simulink model "AFC2_F_trainscg_15_15_15_15_controller_ep_500_Nor_20250717"  (R2021a)
settings: Solver=VariableStepAuto  StartTime=0.0  StopTime=10.0  RelTol=1e-3
libraries: neural x66
(part 3 of 3)

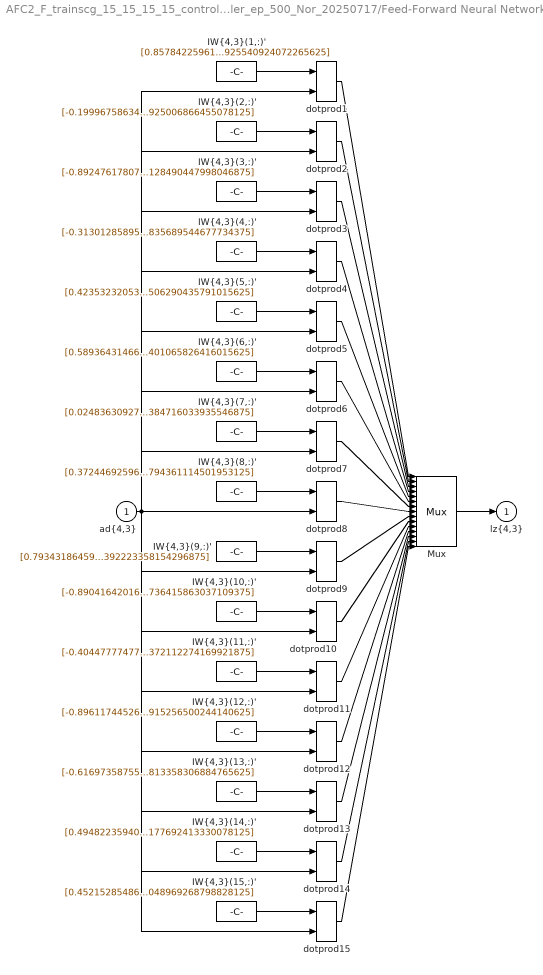
== system AFC2_F_trainscg_15_15_15_15_controller_ep_500_Nor_20250717/Feed-Forward Neural Network/Layer 4/LW{4,3} ==
  "ad{4,3}" : Inport  PortDimensions=15
      mask Display: e = 0.06;c1 = [120 230 180]/255;c2 = ([120 230 180]+0)/(256+128);c3 = ([120 230 180]+128)/(256+128);patch([0 1 1 0],[0 0 1 1],c1);patch([0 1 1 1-e 1-e 0+e],[0 0 1 1-e 0+e 0+e],c2);patch([0 0 1 1-e 0+e 0+e],[0 1 1 1-e 1-e 0+e],c3);plot([0 1 1 0 0],[0 0 1 1 0]);
  "IW{4,3}(1,:)'" : Constant  Value=[0.85784225961529048110065787113853730261325836181640625;0.755479109208128551955496732261963188648223876953125;0.050445139131901829687709692962016561068594455718994140625;-0.426758953537573315628605996607802808284759521484375;0.68113585156923750485447044411557726562023162841796875;0.548222043336579201167069186340086162090301513671875;-0.09920996923674353651367852080511511303484439849853515625;-0.210186876811422396205131235547014512121677398681640625;-0.7277467957558354516578447146457619965076446533203125;0.654091436703768014382376350113190710544586181640625;0.9937004291498972019525126597727648913860321044921875;0.862223254974441299935961069422774016857147216796875;0.4407088843135629208092041153577156364917755126953125;-0.1026007594675311385135074715435621328651905059814453125;0.33596462844713192996692896485910750925540924072265625]
      mask Display: e = 0.06;c1 = [120 150 230]/255;c2 = ([120 150 230]+0)/383;c3 = ([120 150 230]+128)/383;patch([0 1 1 0],[0 0 1 1],c1);patch([0 1 1 1-e 1-e 0+e],[0 0 1 1-e 0+e 0+e],c2);patch([0 0 1 1-e 0+e 0+e],[0 1 1 1-e 1-e 0+e],c3);plot([0 1 1 0 0],[0 0 1 1 0]);disp('weights');
  "IW{4,3}(10,:)'" : Constant  Value=[-0.8904164201605351269819266235572285950183868408203125;0.67793926298775630812087911181151866912841796875;-0.732992210954486633767146486206911504268646240234375;-0.948285057833720745890104808495379984378814697265625;-0.85589678168697302940159943318576551973819732666015625;0.76567535318746748895790688038687221705913543701171875;-0.1853631538863742544975821147090755403041839599609375;0.768810196191384687125491836923174560070037841796875;-0.20373816257141508234695947976433672010898590087890625;-0.80925461474435689268602800439111888408660888671875;-0.127630088537103336676636899937875568866729736328125;-0.5958498069031368249426350303110666573047637939453125;0.46277413232386610530966208898462355136871337890625;-0.89931988538168672331352127002901397645473480224609375;-0.6949987259950594076229890561080537736415863037109375]
      mask Display: e = 0.06;c1 = [120 150 230]/255;c2 = ([120 150 230]+0)/383;c3 = ([120 150 230]+128)/383;patch([0 1 1 0],[0 0 1 1],c1);patch([0 1 1 1-e 1-e 0+e],[0 0 1 1-e 0+e 0+e],c2);patch([0 0 1 1-e 0+e 0+e],[0 1 1 1-e 1-e 0+e],c3);plot([0 1 1 0 0],[0 0 1 1 0]);disp('weights');
  "IW{4,3}(11,:)'" : Constant  Value=[-0.404477774774269993596220729159540496766567230224609375;-0.1346711516861960056257174755955929867923259735107421875;-1.0044851640110368240499383318820036947727203369140625;-0.10694362204521722092831481631947099231183528900146484375;-0.219228550864126792152575262662139721214771270751953125;0.784925570810754980044521289528347551822662353515625;-0.4494260973686199367449489727732725441455841064453125;0.408791248658470995902547429068363271653652191162109375;-0.0217524709232971014127855369224562309682369232177734375;-0.70697111014115987526196249746135435998439788818359375;0.65325901323778357010496620205231010913848876953125;-0.0922130686389561748939058816176839172840118408203125;-0.2799379158284567292724887010990642011165618896484375;-0.56685462762244764878261094054323621094226837158203125;-0.96075786646883187813728000037372112274169921875]
      mask Display: e = 0.06;c1 = [120 150 230]/255;c2 = ([120 150 230]+0)/383;c3 = ([120 150 230]+128)/383;patch([0 1 1 0],[0 0 1 1],c1);patch([0 1 1 1-e 1-e 0+e],[0 0 1 1-e 0+e 0+e],c2);patch([0 0 1 1-e 0+e 0+e],[0 1 1 1-e 1-e 0+e],c3);plot([0 1 1 0 0],[0 0 1 1 0]);disp('weights');
  "IW{4,3}(12,:)'" : Constant  Value=[-0.89611744526934866694745096538099460303783416748046875;-0.05990124759827260281230820737619069404900074005126953125;0.11155310785038198562180156159229227341711521148681640625;0.292599689876200608207312825470580719411373138427734375;0.301985443034309575249807267027790658175945281982421875;0.0822405223753759628824155925030936487019062042236328125;0.433314698716638968534198284032754600048065185546875;-0.9856862277475759714917558085289783775806427001953125;0.30650451235397735416654541040770709514617919921875;0.27569206039626925619501207620487548410892486572265625;-0.21093063153393298847504411241970956325531005859375;-0.1441781603596583583026813357719220221042633056640625;-0.09332817707907252458010560758339124731719493865966796875;0.60984306977241542480072666876367293298244476318359375;-0.133728085119795780943974250476458109915256500244140625]
      mask Display: e = 0.06;c1 = [120 150 230]/255;c2 = ([120 150 230]+0)/383;c3 = ([120 150 230]+128)/383;patch([0 1 1 0],[0 0 1 1],c1);patch([0 1 1 1-e 1-e 0+e],[0 0 1 1-e 0+e 0+e],c2);patch([0 0 1 1-e 0+e 0+e],[0 1 1 1-e 1-e 0+e],c3);plot([0 1 1 0 0],[0 0 1 1 0]);disp('weights');
  "IW{4,3}(13,:)'" : Constant  Value=[-0.6169735875510138356503375689499080181121826171875;0.12196946325811171274455801949443412013351917266845703125;-0.394484793782070075618406690409756265580654144287109375;0.042406510402860718433881714872768498025834560394287109375;0.88124737799676766680789796737371943891048431396484375;0.21174326427215739432341479187016375362873077392578125;-0.433210125755401354030738048095372505486011505126953125;0.36155480448124122094810672933817841112613677978515625;0.8992327827721648958458899869583547115325927734375;0.71234708636273236237457240349613130092620849609375;0.226949763410523974727084350888617336750030517578125;0.93210549922399810185424939845688641071319580078125;-0.2258655976427387523930434554131352342665195465087890625;-0.93860108197167602117616524992627091705799102783203125;0.66555016185605231360256084371940232813358306884765625]
      mask Display: e = 0.06;c1 = [120 150 230]/255;c2 = ([120 150 230]+0)/383;c3 = ([120 150 230]+128)/383;patch([0 1 1 0],[0 0 1 1],c1);patch([0 1 1 1-e 1-e 0+e],[0 0 1 1-e 0+e 0+e],c2);patch([0 0 1 1-e 0+e 0+e],[0 1 1 1-e 1-e 0+e],c3);plot([0 1 1 0 0],[0 0 1 1 0]);disp('weights');
  "IW{4,3}(14,:)'" : Constant  Value=[0.49482235940801666540522774084820412099361419677734375;-0.4633443699893644573961637433967553079128265380859375;0.8250812426062681392835429505794309079647064208984375;-0.25538462229765335198550246786908246576786041259765625;0.471927834000104462486291367895319126546382904052734375;-0.90296620984852771218953648713068105280399322509765625;0.79233153905017028595381134437047876417636871337890625;-0.2246600162756056950907890268354094587266445159912109375;0.450286481803449323280119642731733620166778564453125;1.065736521854187213165232606115750968456268310546875;0.63728147016441827332755565294064581394195556640625;0.240110108266947452904105375637300312519073486328125;0.54537100983026076672643966958275996148586273193359375;0.49952096707471638215025677709490992128849029541015625;0.2023225447090571116337542889596079476177692413330078125]
      mask Display: e = 0.06;c1 = [120 150 230]/255;c2 = ([120 150 230]+0)/383;c3 = ([120 150 230]+128)/383;patch([0 1 1 0],[0 0 1 1],c1);patch([0 1 1 1-e 1-e 0+e],[0 0 1 1-e 0+e 0+e],c2);patch([0 0 1 1-e 0+e 0+e],[0 1 1 1-e 1-e 0+e],c3);plot([0 1 1 0 0],[0 0 1 1 0]);disp('weights');
  "IW{4,3}(15,:)'" : Constant  Value=[0.4521528548690147975008812863961793482303619384765625;0.498047205681803717425282229669392108917236328125;0.9807228794230840041024066522368229925632476806640625;0.87426933268312456704052237910218536853790283203125;-0.034445771129767828455658928987759281881153583526611328125;0.7903040721398146839504761373973451554775238037109375;0.653157784627120374665310009731911122798919677734375;-0.133542756460722056299772475540521554648876190185546875;-0.15248315354482377959044470117078162729740142822265625;0.1597864707538303452594163900357671082019805908203125;0.7724700781252129555554120088345371186733245849609375;0.3907799038360071364195391652174293994903564453125;0.4685422113718786807368132940609939396381378173828125;-0.84392316757664620485712703157332725822925567626953125;0.040266212651737638694715570863991160877048969268798828125]
      mask Display: e = 0.06;c1 = [120 150 230]/255;c2 = ([120 150 230]+0)/383;c3 = ([120 150 230]+128)/383;patch([0 1 1 0],[0 0 1 1],c1);patch([0 1 1 1-e 1-e 0+e],[0 0 1 1-e 0+e 0+e],c2);patch([0 0 1 1-e 0+e 0+e],[0 1 1 1-e 1-e 0+e],c3);plot([0 1 1 0 0],[0 0 1 1 0]);disp('weights');
  "IW{4,3}(2,:)'" : Constant  Value=[-0.1999675863494781713480819007600075565278530120849609375;0.164304483540531898189129833554034121334552764892578125;0.294920972712406748161839686872554011642932891845703125;0.60163861334048807094632138614542782306671142578125;0.689838390875554097192434710450470447540283203125;-0.1725769714967674561822974510505446232855319976806640625;-0.588657896836348282221251793089322745800018310546875;-0.01143321893140521704201884034546310431323945522308349609375;0.62470927507009055279496578805265016853809356689453125;-0.731227381749264271348920374293811619281768798828125;0.1070831469910651367882792328600771725177764892578125;-0.61843070398175559176934257266111671924591064453125;-0.30635878824157902755587201681919395923614501953125;0.371878731756418778875428188257501460611820220947265625;-0.00077214337368226274201099545990700789843685925006866455078125]
      mask Display: e = 0.06;c1 = [120 150 230]/255;c2 = ([120 150 230]+0)/383;c3 = ([120 150 230]+128)/383;patch([0 1 1 0],[0 0 1 1],c1);patch([0 1 1 1-e 1-e 0+e],[0 0 1 1-e 0+e 0+e],c2);patch([0 0 1 1-e 0+e 0+e],[0 1 1 1-e 1-e 0+e],c3);plot([0 1 1 0 0],[0 0 1 1 0]);disp('weights');
  "IW{4,3}(3,:)'" : Constant  Value=[-0.89247617807962276170741233727312646806240081787109375;-0.86100607739435730536570190452039241790771484375;-0.419841694707571988498528980926494114100933074951171875;0.79221535087837258171106213922030292451381683349609375;-0.2607743664207731182358429578016512095928192138671875;0.941656695538196419903442802024073898792266845703125;0.7993019809456687330140312042203731834888458251953125;0.369587645665073905032471657250425778329372406005859375;-0.395000547100446908199700146724353544414043426513671875;-0.88802182418189712365119703463278710842132568359375;0.030916909680651638581139195594005286693572998046875;-0.482835497162455329345220889081247150897979736328125;0.03380749306426929223778898858654429204761981964111328125;0.84153428281462883120411788695491850376129150390625;-0.5796887383710351837606822300585918128490447998046875]
      mask Display: e = 0.06;c1 = [120 150 230]/255;c2 = ([120 150 230]+0)/383;c3 = ([120 150 230]+128)/383;patch([0 1 1 0],[0 0 1 1],c1);patch([0 1 1 1-e 1-e 0+e],[0 0 1 1-e 0+e 0+e],c2);patch([0 0 1 1-e 0+e 0+e],[0 1 1 1-e 1-e 0+e],c3);plot([0 1 1 0 0],[0 0 1 1 0]);disp('weights');
  "IW{4,3}(4,:)'" : Constant  Value=[-0.31301285895226749200759286395623348653316497802734375;0.85004642369605420970657405632664449512958526611328125;-0.6971020802553307138538229992263950407505035400390625;0.1950664900871264817450168038703850470483303070068359375;0.2070968237721194371570021530715166591107845306396484375;1.0010743549489260484364194780937395989894866943359375;0.5251710787464538565672000913764350116252899169921875;0.68577610833234003973046810642699711024761199951171875;-0.48133678245497069081437757631647400557994842529296875;-0.8315058953706808697603491964400745928287506103515625;-0.3386358680194658798967566326609812676906585693359375;0.7957313696805983216364666077424772083759307861328125;0.1133892640242037952447162751923315227031707763671875;0.59421402291022207275972277784603647887706756591796875;0.1432314508081782289394823237671516835689544677734375]
      mask Display: e = 0.06;c1 = [120 150 230]/255;c2 = ([120 150 230]+0)/383;c3 = ([120 150 230]+128)/383;patch([0 1 1 0],[0 0 1 1],c1);patch([0 1 1 1-e 1-e 0+e],[0 0 1 1-e 0+e 0+e],c2);patch([0 0 1 1-e 0+e 0+e],[0 1 1 1-e 1-e 0+e],c3);plot([0 1 1 0 0],[0 0 1 1 0]);disp('weights');
  "IW{4,3}(5,:)'" : Constant  Value=[0.423532320530276729098062560296966694295406341552734375;0.5994190748139638369451631660922430455684661865234375;-0.149139137079837669208615125171490944921970367431640625;0.76802951129515850681173105840571224689483642578125;0.6884912802328846392896366523928008973598480224609375;0.66321777623028455028730832054861821234226226806640625;0.764972614800595973605368271819315850734710693359375;0.17128163825504449935266393367783166468143463134765625;-0.450420586012070078840707765266415663063526153564453125;-0.6912346804131728195130790481925942003726959228515625;-0.139996403213207276650109633919782936573028564453125;0.1867237207722178826685421881848014891147613525390625;-0.687009561771910970406906926655210554599761962890625;0.391552682266078144746046518775983713567256927490234375;-0.75476930316581614111015596790821291506290435791015625]
      mask Display: e = 0.06;c1 = [120 150 230]/255;c2 = ([120 150 230]+0)/383;c3 = ([120 150 230]+128)/383;patch([0 1 1 0],[0 0 1 1],c1);patch([0 1 1 1-e 1-e 0+e],[0 0 1 1-e 0+e 0+e],c2);patch([0 0 1 1-e 0+e 0+e],[0 1 1 1-e 1-e 0+e],c3);plot([0 1 1 0 0],[0 0 1 1 0]);disp('weights');
  "IW{4,3}(6,:)'" : Constant  Value=[0.589364314667610411646592183387838304042816162109375;-0.4281062871592735685766228925785981118679046630859375;-0.2750814383625079795336887400480918586254119873046875;0.88746308239158278041713856509886682033538818359375;0.86700321701421056985736868227832019329071044921875;-0.2222324481751429825493460157304070889949798583984375;-0.4300995639503575329598561438615433871746063232421875;0.1494743217128160495121846906840801239013671875;-0.24861571998082343526448312331922352313995361328125;-0.351560159411901995696325684548355638980865478515625;-0.0163874927925105051684795398614369332790374755859375;0.0076801636936958406209896565997041761875152587890625;0.1241120911235495949398455195478163659572601318359375;-0.781331520951308533540213829837739467620849609375;0.342332465977305933080288014025427401065826416015625]
      mask Display: e = 0.06;c1 = [120 150 230]/255;c2 = ([120 150 230]+0)/383;c3 = ([120 150 230]+128)/383;patch([0 1 1 0],[0 0 1 1],c1);patch([0 1 1 1-e 1-e 0+e],[0 0 1 1-e 0+e 0+e],c2);patch([0 0 1 1-e 0+e 0+e],[0 1 1 1-e 1-e 0+e],c3);plot([0 1 1 0 0],[0 0 1 1 0]);disp('weights');
  "IW{4,3}(7,:)'" : Constant  Value=[0.0248363092718685181392590521909369272179901599884033203125;0.0887981324634880830881655811026575975120067596435546875;0.63494523170573557990792323835194110870361328125;0.09832708137094652023346696978478576056659221649169921875;0.4971322170728871281397687198477797210216522216796875;0.1245748260428689857537420948574435897171497344970703125;0.34652832367269181812474698745063506066799163818359375;-0.236815899621558079157779275192297063767910003662109375;0.078844710400133022343283073496422730386257171630859375;-0.52511982239588295140464424548554234206676483154296875;-0.8579258321740945714140025302185676991939544677734375;0.225619177671118276151673853746615350246429443359375;0.39622423096519876484222777435206808149814605712890625;0.0293784494319486687297082738723474903963506221771240234375;0.2333234784644419856913799549147370271384716033935546875]
      mask Display: e = 0.06;c1 = [120 150 230]/255;c2 = ([120 150 230]+0)/383;c3 = ([120 150 230]+128)/383;patch([0 1 1 0],[0 0 1 1],c1);patch([0 1 1 1-e 1-e 0+e],[0 0 1 1-e 0+e 0+e],c2);patch([0 0 1 1-e 0+e 0+e],[0 1 1 1-e 1-e 0+e],c3);plot([0 1 1 0 0],[0 0 1 1 0]);disp('weights');
  "IW{4,3}(8,:)'" : Constant  Value=[0.37244692596808182116774332826025784015655517578125;0.9695524739412195724952425734954886138439178466796875;0.5605916416882192887527480706921778619289398193359375;0.4567736491887133265521470093517564237117767333984375;-0.58644708412978996392439512419514358043670654296875;-0.5066256047238415494149421647307462990283966064453125;0.32855980883610147458284700405783951282501220703125;-0.087150798296506071238809454371221363544464111328125;0.1238403085319534913111283458420075476169586181640625;-0.9766380177393207961955567952827550470829010009765625;0.7754784310654321277667122558341361582279205322265625;0.6388444844637517494589928901405073702335357666015625;-0.1470889285795251577582121171872131526470184326171875;0.1818094608106728404806062826537527143955230712890625;-0.8880476852244190144602953296271152794361114501953125]
      mask Display: e = 0.06;c1 = [120 150 230]/255;c2 = ([120 150 230]+0)/383;c3 = ([120 150 230]+128)/383;patch([0 1 1 0],[0 0 1 1],c1);patch([0 1 1 1-e 1-e 0+e],[0 0 1 1-e 0+e 0+e],c2);patch([0 0 1 1-e 0+e 0+e],[0 1 1 1-e 1-e 0+e],c3);plot([0 1 1 0 0],[0 0 1 1 0]);disp('weights');
  "IW{4,3}(9,:)'" : Constant  Value=[0.79343186459483361350208951989770866930484771728515625;0.4310020488952888140232744262902997434139251708984375;0.328785881364054233255700410154531709849834442138671875;0.15351500838177900565284517142572440207004547119140625;0.2931924924433786383559663590858690440654754638671875;0.55225764662702736540467185477609746158123016357421875;-0.75438493077637824857362147668027319014072418212890625;0.4137709112504219799433258231147192418575286865234375;-0.210316780358878518963905435157357715070247650146484375;0.0866606987824010965848486875984235666692256927490234375;-0.8707328178982631783355827792547643184661865234375;0.063778338985851501519164230558089911937713623046875;0.67151036371426220394909023525542579591274261474609375;-0.107643762194074010807298691361211240291595458984375;-0.8894121680189417400441698191571049392223358154296875]
      mask Display: e = 0.06;c1 = [120 150 230]/255;c2 = ([120 150 230]+0)/383;c3 = ([120 150 230]+128)/383;patch([0 1 1 0],[0 0 1 1],c1);patch([0 1 1 1-e 1-e 0+e],[0 0 1 1-e 0+e 0+e],c2);patch([0 0 1 1-e 0+e 0+e],[0 1 1 1-e 1-e 0+e],c3);plot([0 1 1 0 0],[0 0 1 1 0]);disp('weights');
  Mux : Mux  Inputs=15
      mask Display: e = 0.06;c1 = [120 150 230]/255;c2 = ([120 150 230]+0)/383;c3 = ([120 150 230]+128)/383;patch([0 1 1 0],[0 0 1 1],c1);patch([0 1 1 1-e 1-e 0+e],[0 0 1 1-e 0+e 0+e],c2);patch([0 0 1 1-e 0+e 0+e],[0 1 1 1-e 1-e 0+e],c3);plot([0 1 1 0 0],[0 0 1 1 0]);disp('Mux');
  dotprod{1..15} (15 alike) : neural/Weight Functions/dotprod
  "lz{4,3}" : Outport
      mask Display: e = 0.06;c1 = [120 230 180]/255;c2 = ([120 230 180]+0)/(256+128);c3 = ([120 230 180]+128)/(256+128);patch([0 1 1 0],[0 0 1 1],c1);patch([0 1 1 1-e 1-e 0+e],[0 0 1 1-e 0+e 0+e],c2);patch([0 0 1 1-e 0+e 0+e],[0 1 1 1-e 1-e 0+e],c3);plot([0 1 1 0 0],[0 0 1 1 0]);
  wires:
  "IW{4,3}(1,:)'"/1 -> dotprod1/1
  "ad{4,3}"/1 -> dotprod1/2, dotprod2/2, dotprod3/2, dotprod4/2, dotprod5/2, dotprod6/2, dotprod7/2, dotprod8/2, dotprod9/2, dotprod10/2, dotprod11/2, dotprod12/2, dotprod13/2, dotprod14/2, dotprod15/2
  dotprod1/1 -> Mux/1
  "IW{4,3}(2,:)'"/1 -> dotprod2/1
  dotprod2/1 -> Mux/2
  "IW{4,3}(3,:)'"/1 -> dotprod3/1
  dotprod3/1 -> Mux/3
  "IW{4,3}(4,:)'"/1 -> dotprod4/1
  dotprod4/1 -> Mux/4
  "IW{4,3}(5,:)'"/1 -> dotprod5/1
  dotprod5/1 -> Mux/5
  "IW{4,3}(6,:)'"/1 -> dotprod6/1
  dotprod6/1 -> Mux/6
  "IW{4,3}(7,:)'"/1 -> dotprod7/1
  dotprod7/1 -> Mux/7
  "IW{4,3}(8,:)'"/1 -> dotprod8/1
  dotprod8/1 -> Mux/8
  "IW{4,3}(9,:)'"/1 -> dotprod9/1
  dotprod9/1 -> Mux/9
  "IW{4,3}(10,:)'"/1 -> dotprod10/1
  dotprod10/1 -> Mux/10
  "IW{4,3}(11,:)'"/1 -> dotprod11/1
  dotprod11/1 -> Mux/11
  "IW{4,3}(12,:)'"/1 -> dotprod12/1
  dotprod12/1 -> Mux/12
  "IW{4,3}(13,:)'"/1 -> dotprod13/1
  dotprod13/1 -> Mux/13
  "IW{4,3}(14,:)'"/1 -> dotprod14/1
  dotprod14/1 -> Mux/14
  "IW{4,3}(15,:)'"/1 -> dotprod15/1
  dotprod15/1 -> Mux/15
  Mux/1 -> "lz{4,3}"/1

== system AFC2_F_trainscg_15_15_15_15_controller_ep_500_Nor_20250717/Feed-Forward Neural Network/Layer 5/Delays 1 ==
  "p{5}" : Inport  PortDimensions=15
      mask Display: e = 0.06;c1 = [120 230 180]/255;c2 = ([120 230 180]+0)/(256+128);c3 = ([120 230 180]+128)/(256+128);patch([0 1 1 0],[0 0 1 1],c1);patch([0 1 1 1-e 1-e 0+e],[0 0 1 1-e 0+e 0+e],c2);patch([0 0 1 1-e 0+e 0+e],[0 1 1 1-e 1-e 0+e],c3);plot([0 1 1 0 0],[0 0 1 1 0]);
  mux : Mux  Inputs=1
      mask Display: e = 0.06;c1 = [120 150 230]/255;c2 = ([120 150 230]+0)/383;c3 = ([120 150 230]+128)/383;patch([0 1 1 0],[0 0 1 1],c1);patch([0 1 1 1-e 1-e 0+e],[0 0 1 1-e 0+e 0+e],c2);patch([0 0 1 1-e 0+e 0+e],[0 1 1 1-e 1-e 0+e],c3);plot([0 1 1 0 0],[0 0 1 1 0]);disp('Mux')
  "pd{5,4}" : Outport
      mask Display: e = 0.06;c1 = [120 230 180]/255;c2 = ([120 230 180]+0)/(256+128);c3 = ([120 230 180]+128)/(256+128);patch([0 1 1 0],[0 0 1 1],c1);patch([0 1 1 1-e 1-e 0+e],[0 0 1 1-e 0+e 0+e],c2);patch([0 0 1 1-e 0+e 0+e],[0 1 1 1-e 1-e 0+e],c3);plot([0 1 1 0 0],[0 0 1 1 0]);
  wires:
  "p{5}"/1 -> mux/1
  mux/1 -> "pd{5,4}"/1

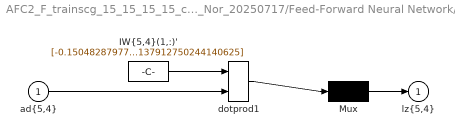
== system AFC2_F_trainscg_15_15_15_15_controller_ep_500_Nor_20250717/Feed-Forward Neural Network/Layer 5/LW{5,4} ==
  "ad{5,4}" : Inport  PortDimensions=15
      mask Display: e = 0.06;c1 = [120 230 180]/255;c2 = ([120 230 180]+0)/(256+128);c3 = ([120 230 180]+128)/(256+128);patch([0 1 1 0],[0 0 1 1],c1);patch([0 1 1 1-e 1-e 0+e],[0 0 1 1-e 0+e 0+e],c2);patch([0 0 1 1-e 0+e 0+e],[0 1 1 1-e 1-e 0+e],c3);plot([0 1 1 0 0],[0 0 1 1 0]);
  "IW{5,4}(1,:)'" : Constant  Value=[-0.150482879779007594489570465157157741487026214599609375;-0.1435557064301314633691930566783412359654903411865234375;0.37469117925264949775510103791020810604095458984375;-0.844238049769963527779736978118307888507843017578125;0.07302774289548906450075804741572937928140163421630859375;0.0339580294124262049848539390950463712215423583984375;-0.80668933393729347347544944568653590977191925048828125;0.87711572866368481271592827397398650646209716796875;-0.0589550060971118783381683670086204074323177337646484375;-0.1187306647285872873709422492538578808307647705078125;0.87433309513333068441198747677844949066638946533203125;-0.0102126581871740777784918208226372371427714824676513671875;0.026582601508947485691169987376270000822842121124267578125;0.78277742528828031520760077910381369292736053466796875;-0.025236072066736593699776136645596125163137912750244140625]
      mask Display: e = 0.06;c1 = [120 150 230]/255;c2 = ([120 150 230]+0)/383;c3 = ([120 150 230]+128)/383;patch([0 1 1 0],[0 0 1 1],c1);patch([0 1 1 1-e 1-e 0+e],[0 0 1 1-e 0+e 0+e],c2);patch([0 0 1 1-e 0+e 0+e],[0 1 1 1-e 1-e 0+e],c3);plot([0 1 1 0 0],[0 0 1 1 0]);disp('weights');
  Mux : Mux  Inputs=1
      mask Display: e = 0.06;c1 = [120 150 230]/255;c2 = ([120 150 230]+0)/383;c3 = ([120 150 230]+128)/383;patch([0 1 1 0],[0 0 1 1],c1);patch([0 1 1 1-e 1-e 0+e],[0 0 1 1-e 0+e 0+e],c2);patch([0 0 1 1-e 0+e 0+e],[0 1 1 1-e 1-e 0+e],c3);plot([0 1 1 0 0],[0 0 1 1 0]);disp('Mux');
  dotprod1 : neural/Weight Functions/dotprod
  "lz{5,4}" : Outport
      mask Display: e = 0.06;c1 = [120 230 180]/255;c2 = ([120 230 180]+0)/(256+128);c3 = ([120 230 180]+128)/(256+128);patch([0 1 1 0],[0 0 1 1],c1);patch([0 1 1 1-e 1-e 0+e],[0 0 1 1-e 0+e 0+e],c2);patch([0 0 1 1-e 0+e 0+e],[0 1 1 1-e 1-e 0+e],c3);plot([0 1 1 0 0],[0 0 1 1 0]);
  wires:
  "IW{5,4}(1,:)'"/1 -> dotprod1/1
  "ad{5,4}"/1 -> dotprod1/2
  dotprod1/1 -> Mux/1
  Mux/1 -> "lz{5,4}"/1
